simulink model "controller1"  (R2025b)
settings: Solver=VariableStepAuto  StartTime=0.0  StopTime=10.0  RelTol=1e-3
settings Model: Creator=Sjoerd  LastModifiedBy=Sjoerd

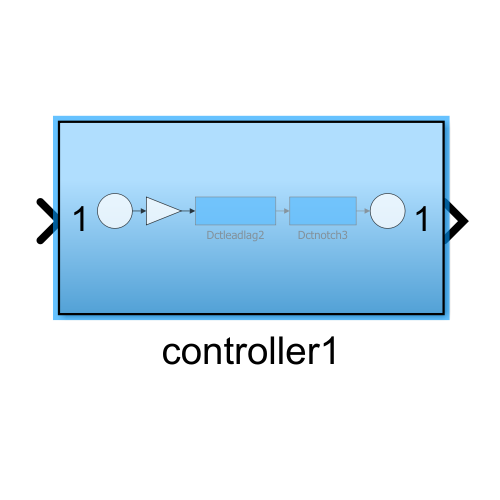
[thumbnail: Simulink's stored preview of the top-level diagram]
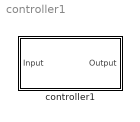
== system controller1 ==
  controller1 : Subsystem

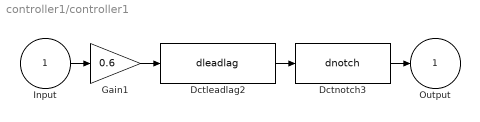
== system controller1/controller1 ==
  Input : Inport
  Dctleadlag2 : S-Function  FunctionName=dleadlag  Parameters=f_num, f_den, 0.001  SFunctionDeploymentMode=off  EnableBusSupport=off  mask(dctools){f_num=5, f_den=25}
      mask prompts: f_num "Zero [Hz]"; f_den "Pole [Hz]"
      mask help: This block implements a discrete time leadlag filter.
      mask Display: disp('DCT leadlag')
  Dctnotch3 : S-Function  FunctionName=dnotch  Parameters=f_num, b_num, f_den, b_den, 0.001  SFunctionDeploymentMode=off  EnableBusSupport=off  mask(dctools){f_num=37, b_num=0.25, f_den=37, b_den=0.5}
      mask prompts: f_num "Zero [Hz]"; b_num "Damping zero [-]"; f_den "Pole [Hz]"; b_den "Damping pole [-]"
      mask help: This block implements a dicrete time 2nd order notch filter.
      mask Display: disp('DCT notch')
  Gain1 : Gain  Gain=0.6
  Output : Outport
  wires:
  Input/1 -> Gain1/1
  Gain1/1 -> Dctleadlag2/1
  Dctleadlag2/1 -> Dctnotch3/1
  Dctnotch3/1 -> Output/1
